simulink model "dubins_path3d_model"  (R2025b)
settings: Solver=VariableStepAuto  StartTime=0.0  StopTime=170.0  MaxStep=1e-2  RelTol=1e-3
InitFcn:
  | init_3dsimulation
StopFcn:
  | export_plot3d
values from neighbouring files (symbols this model uses):
  A = zeros(num, 2)    [init_3dsimulation.m]
  B = zeros(num, 2)    [init_3dsimulation.m]
  C1 = zeros(num, 2)    [init_3dsimulation.m]
  C2 = zeros(num, 2)    [init_3dsimulation.m]
  chi0 = -pi/4    (= -0.785398163397)    [init_3dsimulation.m]
  gamma0 = 0    [init_3dsimulation.m]
  gamma_const = zeros(0, num)    [init_3dsimulation.m]
  goalPose = midPoint - [0, offset, 0]; goalPose(:, 4) = chiF    [init_3dsimulation.m]
  midPoint = (wallTL + wallTR + wallBR + wallBL) ./ 4    [init_3dsimulation.m]
  offset = 30    [init_3dsimulation.m]
  r = 25    [init_3dsimulation.m]
  sign1 = zeros(0, num)    [init_3dsimulation.m]
  sign2 = zeros(0, num)    [init_3dsimulation.m]
  Va = 5    [init_3dsimulation.m]
  x0 = 0    [init_3dsimulation.m]
  y0 = 0    [init_3dsimulation.m]
  z0 = 0    [init_3dsimulation.m]
undefined symbols (not defined in the file or in its folder): num
settings Model: Creator=Parth Bhardwaj  LastModifiedBy=parthbhardwaj

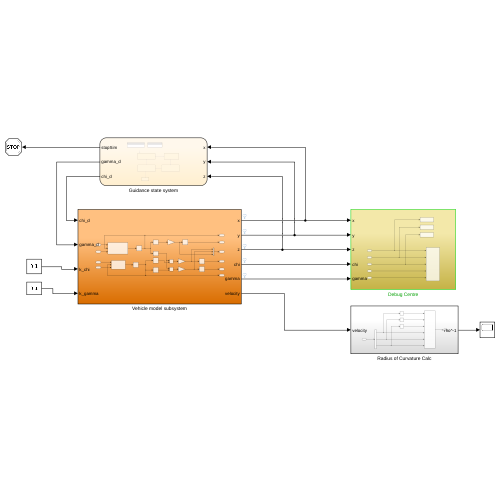
[thumbnail: Simulink's stored preview of the top-level diagram]
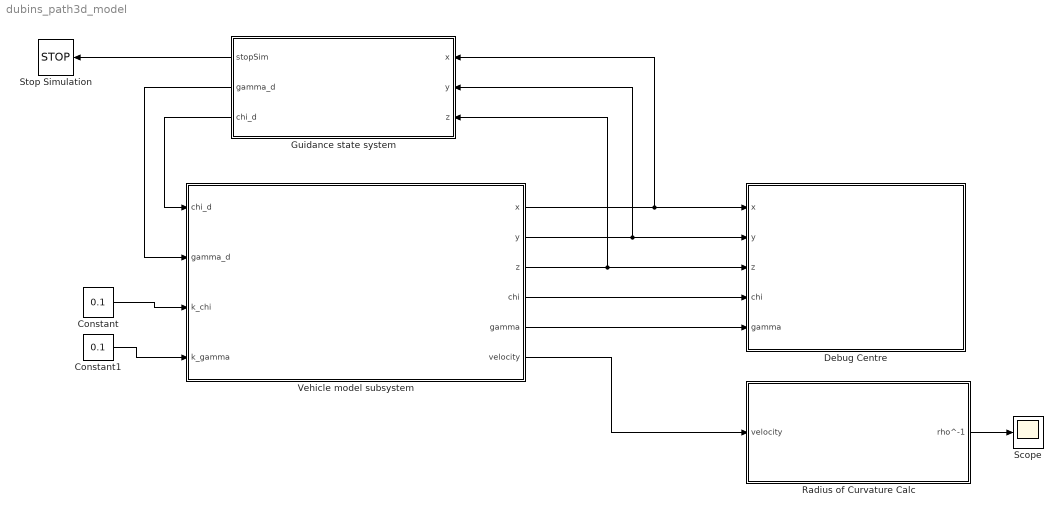
== system dubins_path3d_model ==
  Constant : Constant  Value=0.1
  Constant1 : Constant  Value=0.1
  Debug Centre : Subsystem
  Guidance state system : Stateflow chart  TreatAsAtomicUnit=on
  Radius of Curvature Calc : Subsystem
  Scope : Scope
      settings: ActiveDisplayYMinimum=-0.00508  ActiveDisplayYMaximum=0.04574
  Stop Simulation : Stop
  Vehicle model subsystem : Subsystem
  wires:
  Constant/1 -> Vehicle model subsystem/3(k_chi)
  Vehicle model subsystem/2(y) -> Guidance state system/2(y), Debug Centre/2(y)
  Vehicle model subsystem/4(chi) -> Debug Centre/4(chi)
  Vehicle model subsystem/1(x) -> Guidance state system/1(x), Debug Centre/1(x)
  Vehicle model subsystem/3(z) -> Debug Centre/3(z), Guidance state system/3(z)
  Constant1/1 -> Vehicle model subsystem/4(k_gamma)
  Vehicle model subsystem/5(gamma) -> Debug Centre/5(gamma)
  Guidance state system/3(chi_d) -> Vehicle model subsystem/1(chi_d)
  Guidance state system/2(gamma_d) -> Vehicle model subsystem/2(gamma_d)
  Guidance state system/1(stopSim) -> Stop Simulation/1
  Vehicle model subsystem/6(velocity) -> Radius of Curvature Calc/1(velocity)
  Radius of Curvature Calc/1(rho^-1) -> Scope/1

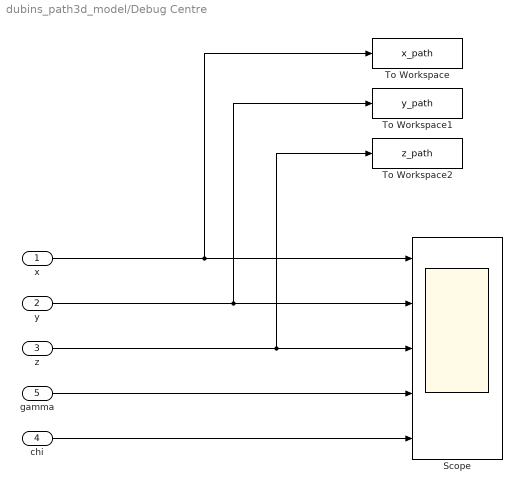
== system dubins_path3d_model/Debug Centre ==
  x : Inport
  y : Inport  Port=2
  z : Inport  Port=3
  chi : Inport  Port=4
  gamma : Inport  Port=5
  Scope : Scope  NumInputPorts=5
      settings: ActiveDisplayYMinimum=-15.33373  ActiveDisplayYMaximum=9.82719
  To Workspace : ToWorkspace  VariableName=x_path  SampleTime=-1
      settings: Save2DSignal=2-D array (concatenate along first dimension)
  To Workspace1 : ToWorkspace  VariableName=y_path  SampleTime=-1
      settings: Save2DSignal=2-D array (concatenate along first dimension)
  To Workspace2 : ToWorkspace  VariableName=z_path  SampleTime=-1
      settings: Save2DSignal=2-D array (concatenate along first dimension)
  wires:
  x/1 -> To Workspace/1, Scope/1
  y/1 -> To Workspace1/1, Scope/2
  chi/1 -> Scope/5
  z/1 -> To Workspace2/1, Scope/3
  gamma/1 -> Scope/4

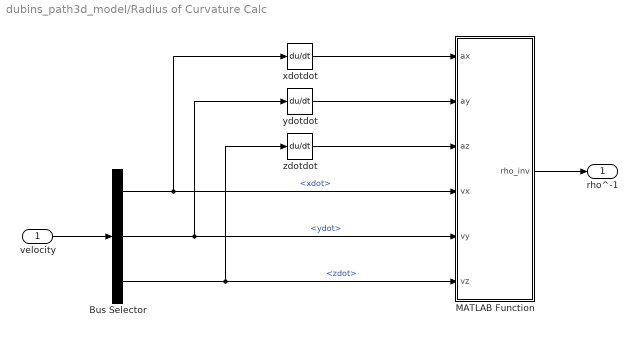
== system dubins_path3d_model/Radius of Curvature Calc ==
  velocity : Inport
  Bus Selector : BusSelector  OutputSignals=xdot,ydot,zdot
  MATLAB Function : MATLAB Function  TreatAsAtomicUnit=on
  xdotdot : Derivative
  ydotdot : Derivative
  zdotdot : Derivative
  rho^-1 : Outport
  wires:
  velocity/1 -> Bus Selector/1
  Bus Selector/3 -> zdotdot/1, MATLAB Function/6(vz)  "<zdot>"
  ydotdot/1 -> MATLAB Function/2(ay)
  xdotdot/1 -> MATLAB Function/1(ax)
  zdotdot/1 -> MATLAB Function/3(az)
  Bus Selector/1 -> xdotdot/1, MATLAB Function/4(vx)  "<xdot>"
  Bus Selector/2 -> ydotdot/1, MATLAB Function/5(vy)  "<ydot>"
  MATLAB Function/1(rho_inv) -> rho^-1/1

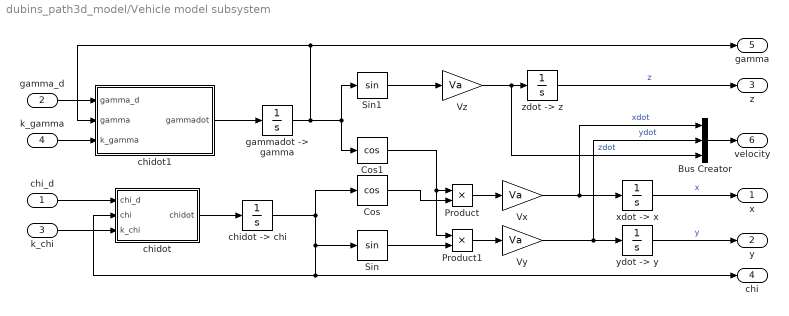
== system dubins_path3d_model/Vehicle model subsystem ==
  chi_d : Inport
  gamma_d : Inport  Port=2
  k_chi : Inport  Port=3
  k_gamma : Inport  Port=4
  Bus Creator : BusCreator  Inputs=3
  Cos : Trigonometry  Operator=cos
  Cos1 : Trigonometry  Operator=cos
  Product : Product
  Product1 : Product
  Sin : Trigonometry
  Sin1 : Trigonometry
  Vx : Gain  Gain=Va
  Vy : Gain  Gain=Va
  Vz : Gain  Gain=Va
  chidot : MATLAB Function  TreatAsAtomicUnit=on
  "chidot -> chi" : Integrator  InitialCondition=chi0
  chidot1 : MATLAB Function  TreatAsAtomicUnit=on
  "gammadot -> gamma" : Integrator  InitialCondition=gamma0
  "xdot -> x" : Integrator  InitialCondition=x0
  "ydot -> y" : Integrator  InitialCondition=y0
  "zdot -> z" : Integrator  InitialCondition=z0
  x : Outport
  y : Outport  Port=2
  z : Outport  Port=3
  chi : Outport  Port=4
  gamma : Outport  Port=5
  velocity : Outport  Port=6
  wires:
  chidot/1(chidot) -> "chidot -> chi"/1
  Vx/1 -> Bus Creator/1, "xdot -> x"/1  "xdot"
  Vy/1 -> Bus Creator/2, "ydot -> y"/1  "ydot"
  "ydot -> y"/1 -> y/1  "y"
  "xdot -> x"/1 -> x/1  "x"
  k_chi/1 -> chidot/3(k_chi)
  chi_d/1 -> chidot/1(chi_d)
  k_gamma/1 -> chidot1/3(k_gamma)
  gamma_d/1 -> chidot1/1(gamma_d)
  chidot1/1(gammadot) -> "gammadot -> gamma"/1
  "gammadot -> gamma"/1 -> gamma/1, chidot1/2(gamma), Sin1/1, Cos1/1
  "chidot -> chi"/1 -> chidot/2(chi), chi/1, Sin/1, Cos/1
  Cos/1 -> Product/2
  Cos1/1 -> Product1/1, Product/1
  Sin/1 -> Product1/2
  Product/1 -> Vx/1
  Product1/1 -> Vy/1
  Sin1/1 -> Vz/1
  Vz/1 -> Bus Creator/3, "zdot -> z"/1  "zdot"
  "zdot -> z"/1 -> z/1  "z"
  Bus Creator/1 -> velocity/1

== matlab function dubins_path3d_model/Vehicle model subsystem/chidot1 ==
  data: gamma_d input; gammadot output; gamma input; k_gamma input
function gammadot = fcn(gamma_d, gamma, k_gamma)
    gammadot = k_gamma * atan2(sin(gamma_d - gamma), cos(gamma_d - gamma));
end

== matlab function dubins_path3d_model/Vehicle model subsystem/chidot ==
  data: chi_d input; chidot output; chi input; k_chi input
function chidot = fcn(chi_d, chi, k_chi)
    chidot = k_chi * atan2(sin(chi_d - chi), cos(chi_d - chi));
end

== stateflow chart dubins_path3d_model/Guidance state system ==
  state Arc1
    entry:
    lambda = sign1(i) * pi/36;
    EA = atan2(A(i,2) - C1(i,2), A(i,1) - C1(i,1));
    AFC = atan2(y - C1(i,2), x - C1(i,1));
    value = (mod(EA - AFC, 2*pi) - pi) * sign1(i);
    during:
    [chi_d, gamma_d] = carrot_circle(x, y, z, C1(i,1:2), r, lambda, gamma_const(i));
    AFC = atan2(y - C1(i,2), x - C1(i,1));
    value = (mod(EA - AFC, 2*pi) - pi) * sign1(i);
  state straight
    entry:
    delta = 4.5;
    StDist = norm(B(i,1:3) - A(i,1:3));
    [chi_d, R, gamma_d] = carrot_st(x, y, z, A(i,1:3), B(i,1:3), delta);
    during:
    [chi_d, R, gamma_d] = carrot_st(x, y, z, A(i,1:3), B(i,1:3), delta);
  state straight1
    entry:
    delta = 4.5;
    i = i+1
    StDist = offset;
    [chi_d, R, gamma_d] = carrot_st(x, y, z, goalPose(i-1,1:3),midPoint(i-1,1:3), delta);
    during:
    [chi_d, R, gamma_d] = carrot_st(x, y, z, goalPose(i-1,1:3),midPoint(i-1,1:3), delta);
  state Arc2
    entry:
    lambda = sign2(i) * pi/36;
    EA = atan2(goalPose(i,2) - C2(i,2), goalPose(i,1) - C2(i,1));
    AFC = atan2(y - C2(i,2), x - C2(i,1));
    value = (mod(EA - AFC, 2*pi) - pi) * sign2(i);
    during:
    [chi_d, gamma_d] = carrot_circle(x, y, z, C2(i,1:2), r, lambda, gamma_const(i));
    AFC = atan2(y - C2(i,2), x - C2(i,1));
    value = (mod(EA - AFC, 2*pi) - pi) * sign2(i);
  state stop
    entry:
    stopSim = 1;
  (default) -> Arc1 : {i = 1;}
  Arc1 -> straight : [value < -pi/12]
  straight1 -> Arc1 [order 2] : [StDist - R - delta < 0]
  straight -> Arc2 : [StDist - R - delta < 0]
  Arc2 -> straight1 : [value < -pi/12]
  straight1 -> stop [order 1] : [StDist - R - delta < 0 && i > num]
  data: xf function_input; yf function_input; zf function_input; chi_df function_output; gamma_df function_output; C function_input; rf function_input; lambdaf function_input; gamma_constf function_input; xf function_input; yf function_input; zf function_input; W_i function_input; W_f function_input; deltaf function_input; chi_df function_output; Rf function_output; gamma_df function_output; stopSim output =0; x input; y input; gamma_d output; chi_d output; A parameter; z input; Ru local; B parameter; R local; StDist local; delta local; r parameter; sign1 parameter; AFC local; EA local; lambda local; value local; C1 parameter; gamma_const parameter; sign2 parameter; offset parameter; goalPose parameter; C2 parameter; midPoint parameter; i local; num parameter
  function [chi_df, gamma_df] = carrot_circle(xf, yf, zf, C, rf, lambdaf, gamma_constf):
    | function [chi_df, gamma_df] = carrot_circle(xf, yf, zf, C, rf, lambdaf, gamma_constf)
    |     
    |     theta = atan2(yf - C(2), xf - C(1));
    |     x_t = C(1) + rf * cos(theta + lambdaf);
    |     y_t = C(2) + rf * sin(theta + lambdaf);
    |     z_t = rf * lambdaf * tan(gamma_constf);
    |     chi_df = atan2(y_t - yf, x_t - xf);
    |     gamma_df = asin((z_t - zf) / norm([xf,yf,zf] - [x_t,y_t,z_t]));
    | end
  function [chi_df, Rf, gamma_df] = carrot_st(xf, yf, zf, W_i, W_f, deltaf):
    | function [chi_df, Rf, gamma_df] = carrot_st(xf, yf, zf, W_i, W_f, deltaf)
    | 
    |     Ru = ([xf, yf, zf] - W_i);
    |     b = (W_f - W_i) / norm(W_f - W_i);
    |     Rf = dot(Ru, b);
    |     x_t = W_i(1) + (Rf + deltaf)*b(1); 
    |     y_t = W_i(2) + (Rf + deltaf)*b(2); 
    |     z_t = W_i(3) + (Rf + deltaf)*b(3);
    |     chi_df = atan2(y_t - yf, x_t - xf);
    |     gamma_df = asin((z_t-zf) / norm([x_t, y_t, z_t] - [xf, yf, zf]));
    | 
    | end

== matlab function dubins_path3d_model/Radius of Curvature Calc/MATLAB Function ==
  data: ax input; rho_inv output; ay input; az input; vx input; vy input; vz input
function rho_inv = roc(ax, ay, az, vx, vy, vz)
    
    vel = norm([vx, vy, vz]);
    vel_cross_acc = norm(cross([vx, vy, vz], [ax, ay, az]));
    rho_inv = vel_cross_acc / (vel^3);
end
